simulink model "three_phase_dab"  (R2026a)
settings: Solver=ode23tb  StopTime=param.sim.simlength  FixedStep=tc  MaxStep=param.glb_time.tc
values from neighbouring files (symbols this model uses):
  param = struct()    [init_model.m]
libraries: fl_lib x30, nesl_utility x23, discrete_time_low_pass_filter x6, single_phase_transformer x3, lithium_ion_battery x2, pi_ctrl x2, three_phase_inverter_ideal_switch_based_model x2, three_phase_inverter_mosfet_based_with_thermal_model x2, three_phase_dab_modulator x1
(part 2 of 2)

== system three_phase_dab/dab_modA/dcdc_with_galvanic_isolation/three_phase_inverter_1/three_phase_inverter_1 ==
  inv1_gate_cmds : Inport
  three_phase_inverter_ideal_switch_based_model : three_phase_inverter_ideal_switch_based_model/three phase inverter ideal switch based model  Commented=on  Ron_ideal_switch=param.dab3.ideal_switch.Rds_on  Vth=param.dab3.ideal_switch.Vth  Vgamma=param.dab3.ideal_switch.Vdon_diode  Rdon_diode=param.dab3.ideal_switch.Rdon_diode  Csnubber=param.dab3.ideal_switch.Csnubber  Rsnubber=param.dab3.ideal_switch.Rsnubber
  three_phase_inverter_mosfet_based_with_thermal_model : three_phase_inverter_mosfet_based_with_thermal_model/three phase inverter mosfet based with thermal model  mass_heatsink_m=param.thermal.heatsink.no_weight  specific_heat_m=param.thermal.heatsink.cp  rth_mosfet_HA_m=param.thermal.heatsink.Rth_mosfet_HA  rth_mosfet_JH_m=param.dab3.mosfet.Rth_mosfet_JH  Rds_on_m=param.dab3.mosfet.Rds_on  Vth_m=param.dab3.mosfet.Vth  Eon_m=param.dab3.mosfet.Eon  Eoff_m=param.dab3.mosfet.Eoff  Voff_sw_loss_m=param.dab3.mosfet.Voff_sw_losses  Ion_sw_loss_m=param.dab3.mosfet.Ion_sw_losses  Vdon_diode_m=param.dab3.mosfet.Vdon_diode  Rdon_diode_m=param.dab3.mosfet.Rdon_diode  JunctionTermalMass_m=param.dab3.mosfet.JunctionTermalMass  Tambient_m=param.thermal.heatsink.Tambient  DThs_init_m=param.thermal.heatsink.DThs_init
  udc(+) : PMIOPort  Side=Left
  u : PMIOPort  Port=2  Side=Right
  v : PMIOPort  Port=3  Side=Right
  udc(-) : PMIOPort  Port=4  Side=Left
  w : PMIOPort  Port=5  Side=Right
  tag scope: inverter_1_dab_devices_modA=global
  wires:
  inv1_gate_cmds/1 -> three_phase_inverter_ideal_switch_based_model/1, three_phase_inverter_mosfet_based_with_thermal_model/1
  three_phase_inverter_mosfet_based_with_thermal_model/1 -> [inverter_1_dab_devices_modA]
  connections:
  u/RConn1 -- three_phase_inverter_ideal_switch_based_model/RConn1 -- three_phase_inverter_mosfet_based_with_thermal_model/RConn1
  v/RConn1 -- three_phase_inverter_ideal_switch_based_model/RConn2 -- three_phase_inverter_mosfet_based_with_thermal_model/RConn2
  udc(-)/RConn1 -- three_phase_inverter_ideal_switch_based_model/LConn2 -- three_phase_inverter_mosfet_based_with_thermal_model/LConn2
  w/RConn1 -- three_phase_inverter_ideal_switch_based_model/RConn3 -- three_phase_inverter_mosfet_based_with_thermal_model/RConn3
  udc(+)/RConn1 -- three_phase_inverter_ideal_switch_based_model/LConn1 -- three_phase_inverter_mosfet_based_with_thermal_model/LConn1

== system three_phase_dab/dab_modA/dcdc_with_galvanic_isolation/three_phase_inverter_2/dclink_2 ==
  CFi_dc2 : fl_lib/Electrical/Electrical Elements/Capacitor  c=param.dab3.hw.Cdc_dc2 F  r=param.dab3.hw.RCdc_dc2 Ohm  g=0 1/Ohm  i_specify=off  i_priority=None  i=0 A  i_nominal_specify=off  i_nominal_value=1  i_nominal_unit=A  v_specify=off  v_priority=None  v=0 V  v_nominal_specify=off  v_nominal_value=1  v_nominal_unit=V  vc_specify=on  vc_priority=High  vc=param.dab3.ic.vc_dc2 V  vc_nominal_specify=off  vc_nominal_value=1  vc_nominal_unit=V
  Current Sensor2 : fl_lib/Electrical/Electrical Sensors/Current Sensor
  PS-Simulink Converter6 : nesl_utility/PS-Simulink Converter  PhysicalDomain=network_engine_domain  SubClassName=ps_output  LeftPortType=input  RightPortType=output  PseudoPeriodic=off  Frequencies=[]  VectorFormat=1-D array  Unit=A  AffineConversion=on
  ui_measure : Subsystem
  Udc(+) : PMIOPort  Side=Left
  Udc(-) : PMIOPort  Port=2  Side=Left
  udc(+) : PMIOPort  Port=3  Side=Right
  udc(-) : PMIOPort  Port=4  Side=Right
  tag scope: CFi_dc2_current_modA=global
  wires:
  PS-Simulink Converter6/1 -> [CFi_dc2_current_modA]  "CFi_dc2_current_modA"
  connections:
  CFi_dc2/RConn1 -- Current Sensor2/LConn1
  PS-Simulink Converter6/LConn1 -- Current Sensor2/RConn1
  Current Sensor2/RConn2 -- ui_measure/RConn2 -- Udc(-)/RConn1
  CFi_dc2/LConn1 -- ui_measure/RConn1 -- Udc(+)/RConn1
  ui_measure/LConn2 -- udc(-)/RConn1
  ui_measure/LConn1 -- udc(+)/RConn1

== system three_phase_dab/dab_modA/dcdc_with_galvanic_isolation/three_phase_inverter_2/three_phase_inverter_2 ==
  inv2_gate_cmds : Inport
  three_phase_inverter_ideal_switch_based_model : three_phase_inverter_ideal_switch_based_model/three phase inverter ideal switch based model  Commented=on  Ron_ideal_switch=param.dab3.ideal_switch.Rds_on  Vth=param.dab3.ideal_switch.Vth  Vgamma=param.dab3.ideal_switch.Vdon_diode  Rdon_diode=param.dab3.ideal_switch.Rdon_diode  Csnubber=param.dab3.ideal_switch.Csnubber  Rsnubber=param.dab3.ideal_switch.Rsnubber
  three_phase_inverter_mosfet_based_with_thermal_model : three_phase_inverter_mosfet_based_with_thermal_model/three phase inverter mosfet based with thermal model  mass_heatsink_m=param.thermal.heatsink.no_weight  specific_heat_m=param.thermal.heatsink.cp  rth_mosfet_HA_m=param.thermal.heatsink.Rth_mosfet_HA  rth_mosfet_JH_m=param.dab3.mosfet.Rth_mosfet_JH  Rds_on_m=param.dab3.mosfet.Rds_on  Vth_m=param.dab3.mosfet.Vth  Eon_m=param.dab3.mosfet.Eon  Eoff_m=param.dab3.mosfet.Eoff  Voff_sw_loss_m=param.dab3.mosfet.Voff_sw_losses  Ion_sw_loss_m=param.dab3.mosfet.Ion_sw_losses  Vdon_diode_m=param.dab3.mosfet.Vdon_diode  Rdon_diode_m=param.dab3.mosfet.Rdon_diode  JunctionTermalMass_m=param.dab3.mosfet.JunctionTermalMass  Tambient_m=param.thermal.heatsink.Tambient  DThs_init_m=param.thermal.heatsink.DThs_init
  udc(+) : PMIOPort  Side=Right
  u : PMIOPort  Port=2  Side=Left
  v : PMIOPort  Port=3  Side=Left
  udc(-) : PMIOPort  Port=4  Side=Right
  w : PMIOPort  Port=5  Side=Left
  tag scope: inverter_2_dab_devices_modA=global
  wires:
  inv2_gate_cmds/1 -> three_phase_inverter_ideal_switch_based_model/1, three_phase_inverter_mosfet_based_with_thermal_model/1
  three_phase_inverter_mosfet_based_with_thermal_model/1 -> [inverter_2_dab_devices_modA]
  connections:
  udc(-)/RConn1 -- three_phase_inverter_mosfet_based_with_thermal_model/LConn2 -- three_phase_inverter_ideal_switch_based_model/LConn2
  udc(+)/RConn1 -- three_phase_inverter_mosfet_based_with_thermal_model/LConn1 -- three_phase_inverter_ideal_switch_based_model/LConn1
  u/RConn1 -- three_phase_inverter_ideal_switch_based_model/RConn1 -- three_phase_inverter_mosfet_based_with_thermal_model/RConn1
  w/RConn1 -- three_phase_inverter_ideal_switch_based_model/RConn3 -- three_phase_inverter_mosfet_based_with_thermal_model/RConn3
  v/RConn1 -- three_phase_inverter_ideal_switch_based_model/RConn2 -- three_phase_inverter_mosfet_based_with_thermal_model/RConn2

== system three_phase_dab/dab_modA/dab_ctrl/ui_ctrl1/dab_ctrl/Vout Ctrl ==
  vout_ref : Inport
  vout : Inport  Port=2
  pi_ctrl : pi_ctrl/pi_ctrl  kp=param.dab3.ctrl.kp_udc  ki=param.dab3.ctrl.ki_udc  ts=param.glb_time.ts_dab  lim_up=2  lim_down=-2
  ctrlv_out : Outport
  wires:
  vout_ref/1 -> pi_ctrl/1
  vout/1 -> pi_ctrl/2
  pi_ctrl/1 -> ctrlv_out/1

== system three_phase_dab/dab_modA/dab_ctrl/ui_ctrl1/dab_ctrl/current control ==
  iout_ref : Inport
  iout : Inport  Port=2
  Gain : Gain  Gain=param.dab3.mod.k_ff
  i_out_dab_tracking : Scope  NumInputPorts=3
      settings: ActiveDisplayYMinimum=-1.1373515596021884  ActiveDisplayYMaximum=-0.8283017665059349  DataLoggingVariableName=ScopeData12
  pi_ctrl : pi_ctrl/pi_ctrl  kp=param.dab3.ctrl.kp_idc  ki=param.dab3.ctrl.ki_idc  ts=param.glb_time.ts_dab  lim_up=1  lim_down=-1
  i_ctrl_out : Outport
  wires:
  iout_ref/1 -> pi_ctrl/1, i_out_dab_tracking/1, Gain/1  "i_out_dab_ref"
  iout/1 -> pi_ctrl/2, i_out_dab_tracking/2  "i_out_dab"
  Gain/1 -> pi_ctrl/3
  pi_ctrl/1 -> i_out_dab_tracking/3, i_ctrl_out/1  "i_ctrl_out"

== system three_phase_dab/dab_modA/dab_ctrl/ui_ctrl1/dab_ctrl/rate_limiter ==
  u : Inport
  Constant : Constant  Value=param.dab3.bench.r_rise
  Constant1 : Constant  Value=param.dab3.bench.r_fall
  MATLAB Function : MATLAB Function  TreatAsAtomicUnit=on
  y : Outport
  wires:
  MATLAB Function/1(y) -> y/1
  u/1 -> MATLAB Function/1(u)
  [local_time] -> MATLAB Function/4(t_now)
  Constant/1 -> MATLAB Function/2(r_rise)
  Constant1/1 -> MATLAB Function/3(r_fall)

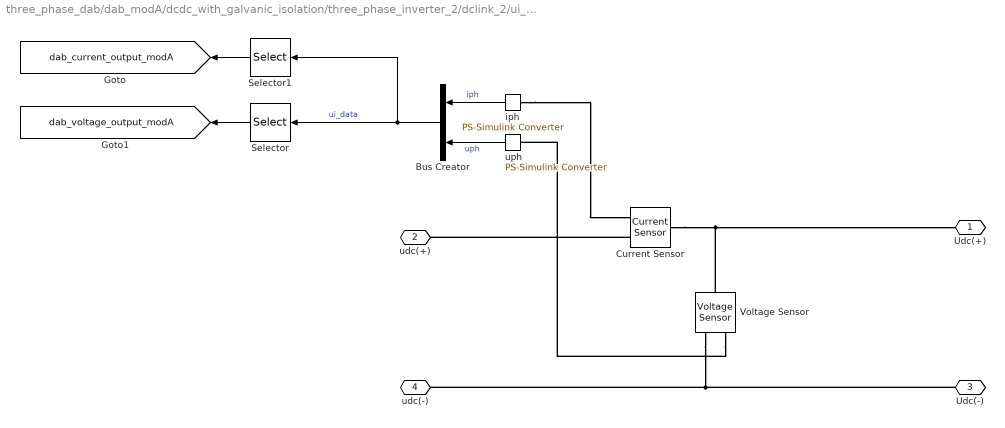
== system three_phase_dab/dab_modA/dcdc_with_galvanic_isolation/three_phase_inverter_2/dclink_2/ui_measure ==
  Bus Creator : BusCreator  Inputs=2
  Current Sensor : fl_lib/Electrical/Electrical Sensors/Current Sensor
  Selector : Selector  InputPortWidth=2  IndexOptions=Index vector (dialog)  Indices=2  OutputSizes=1
  Selector1 : Selector  InputPortWidth=2  IndexOptions=Index vector (dialog)  Indices=1  OutputSizes=1
  Voltage Sensor : fl_lib/Electrical/Electrical Sensors/Voltage Sensor
  iph : nesl_utility/PS-Simulink Converter  PhysicalDomain=network_engine_domain  SubClassName=ps_output  LeftPortType=input  RightPortType=output  PseudoPeriodic=off  Frequencies=[]  VectorFormat=1-D array  Unit=A  AffineConversion=off
  uph : nesl_utility/PS-Simulink Converter  PhysicalDomain=network_engine_domain  SubClassName=ps_output  LeftPortType=input  RightPortType=output  PseudoPeriodic=off  Frequencies=[]  VectorFormat=1-D array  Unit=V  AffineConversion=off
  Udc(+) : PMIOPort  Side=Left
  udc(+) : PMIOPort  Port=2  Side=Right
  Udc(-) : PMIOPort  Port=3  Side=Left
  udc(-) : PMIOPort  Port=4  Side=Right
  tag scope: dab_current_output_modA=global, dab_voltage_output_modA=global
  wires:
  Selector1/1 -> [dab_current_output_modA]
  Selector/1 -> [dab_voltage_output_modA]
  Bus Creator/1 -> Selector/1, Selector1/1  "ui_data"
  iph/1 -> Bus Creator/1  "iph"
  uph/1 -> Bus Creator/2  "uph"
  connections:
  iph/LConn1 -- Current Sensor/RConn1
  Voltage Sensor/LConn1 -- Udc(+)/RConn1 -- Current Sensor/LConn1
  Current Sensor/RConn2 -- udc(+)/RConn1
  Voltage Sensor/RConn1 -- uph/LConn1
  Voltage Sensor/RConn2 -- Udc(-)/RConn1 -- udc(-)/RConn1

== matlab function three_phase_dab/dab_modA/dab_ctrl/ui_ctrl1/dab_ctrl/rate_limiter/MATLAB Function ==
  data: u input; y output; r_rise input; r_fall input; t_now input
function y = rate_limiter(u, r_rise, r_fall, t_now)

persistent y_prev t_prev;

y = u;

if isempty(y_prev)
    y_prev = u;
    t_prev = t_now;
    return;
end

dt = t_now - t_prev;

if dt <= 0
    y = y_prev;
    return;
end

delta = u - y_prev;
d_max =  r_rise * dt;
d_min = -r_fall * dt;

y      = y_prev + max(d_min, min(d_max, delta));
y_prev = y;
t_prev = t_now;
